simulink model "third_lab"  (R2025b)
settings: Solver=VariableStepAuto  StartTime=0.0  StopTime=10.0  RelTol=1e-3
values from neighbouring files (symbols this model uses):
  p1 = 0.001    [lab3.m]
  p2 = 0.072    [lab3.m]
  p3 = 0.05    [lab3.m]
settings Model: Creator=reino  LastModifiedBy=reino

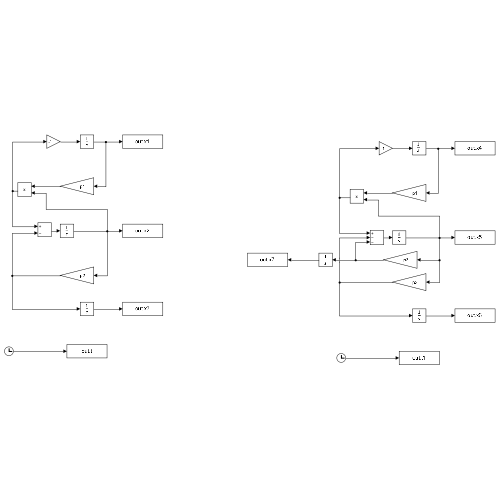
[thumbnail: Simulink's stored preview of the top-level diagram]
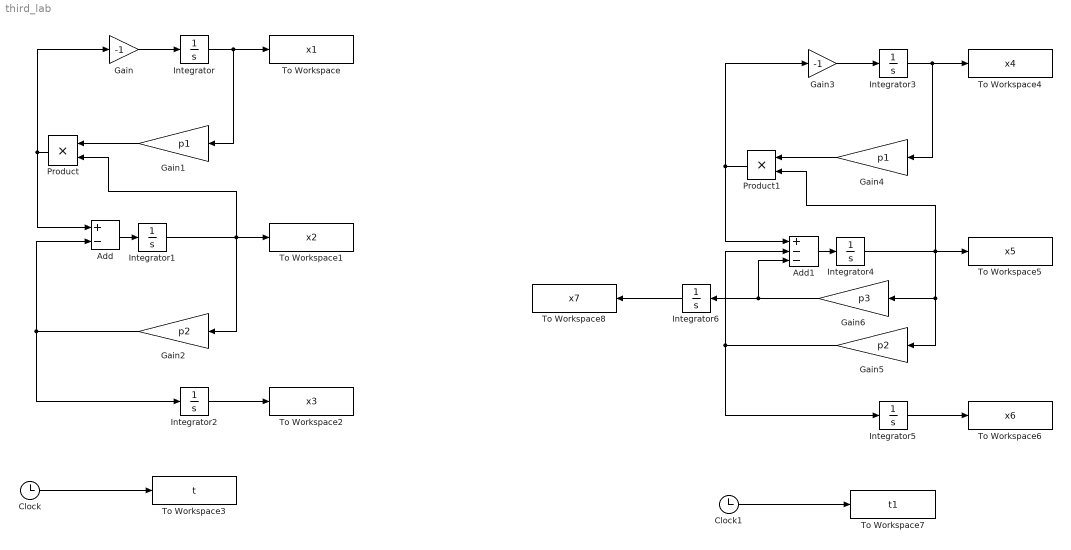
== system third_lab ==
  Add : Sum  Inputs=+-
  Add1 : Sum  Inputs=+--
  Clock : Clock
  Clock1 : Clock
  Gain : Gain  Gain=-1
  Gain1 : Gain  Gain=p1
  Gain2 : Gain  Gain=p2
  Gain3 : Gain  Gain=-1
  Gain4 : Gain  Gain=p1
  Gain5 : Gain  Gain=p2
  Gain6 : Gain  Gain=p3
  Integrator : Integrator  InitialCondition=880
  Integrator1 : Integrator  InitialCondition=20
  Integrator2 : Integrator  InitialCondition=100
  Integrator3 : Integrator  InitialCondition=880
  Integrator4 : Integrator  InitialCondition=20
  Integrator5 : Integrator  InitialCondition=100
  Integrator6 : Integrator
  Product : Product
  Product1 : Product
  To Workspace : ToWorkspace  VariableName=x1  SaveFormat=Timeseries  SampleTime=-1
  To Workspace1 : ToWorkspace  VariableName=x2  SaveFormat=Timeseries  SampleTime=-1
  To Workspace2 : ToWorkspace  VariableName=x3  SaveFormat=Timeseries  SampleTime=-1
  To Workspace3 : ToWorkspace  VariableName=t  SaveFormat=Timeseries  SampleTime=-1
  To Workspace4 : ToWorkspace  VariableName=x4  SaveFormat=Timeseries  SampleTime=-1
  To Workspace5 : ToWorkspace  VariableName=x5  SaveFormat=Timeseries  SampleTime=-1
  To Workspace6 : ToWorkspace  VariableName=x6  SaveFormat=Timeseries  SampleTime=-1
  To Workspace7 : ToWorkspace  VariableName=t1  SaveFormat=Timeseries  SampleTime=-1
  To Workspace8 : ToWorkspace  VariableName=x7  SaveFormat=Timeseries  SampleTime=-1
  wires:
  Integrator/1 -> Gain1/1, To Workspace/1
  Integrator1/1 -> Product/2, Gain2/1, To Workspace1/1
  Integrator2/1 -> To Workspace2/1
  Gain1/1 -> Product/1
  Gain/1 -> Integrator/1
  Product/1 -> Gain/1, Add/1
  Gain2/1 -> Integrator2/1, Add/2
  Add/1 -> Integrator1/1
  Clock/1 -> To Workspace3/1
  Gain5/1 -> Integrator5/1, Add1/2
  Add1/1 -> Integrator4/1
  Clock1/1 -> To Workspace7/1
  Integrator3/1 -> Gain4/1, To Workspace4/1
  Integrator4/1 -> Product1/2, Gain6/1, Gain5/1, To Workspace5/1
  Gain4/1 -> Product1/1
  Product1/1 -> Gain3/1, Add1/1
  Integrator5/1 -> To Workspace6/1
  Gain3/1 -> Integrator3/1
  Integrator6/1 -> To Workspace8/1
  Gain6/1 -> Add1/3, Integrator6/1
